simulink model "ev_battery_soc"  (R2026b)
settings: Solver=VariableStepAuto  StopTime=600
settings Model: Creator=Hassan  LastModifiedBy=Hassan

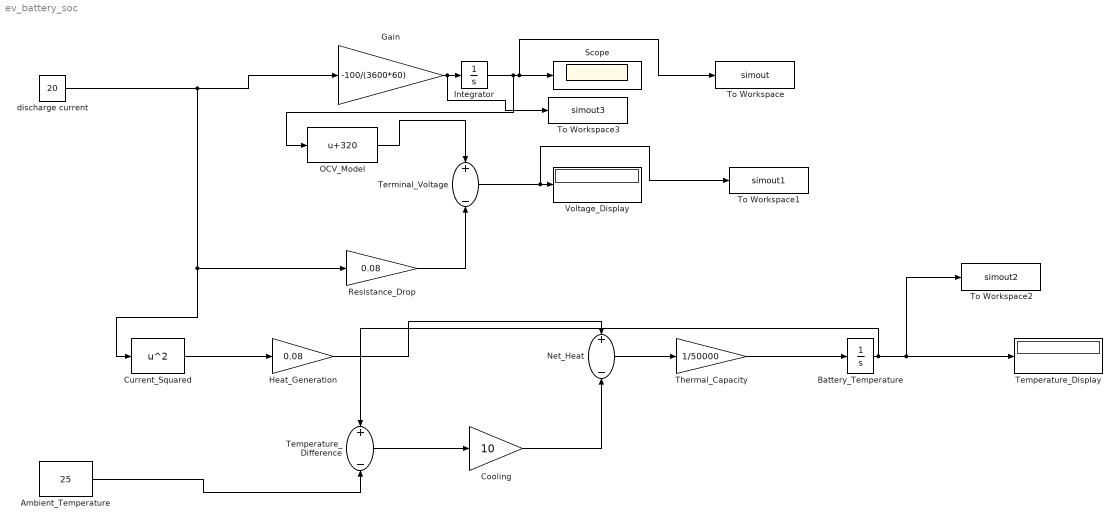
== system ev_battery_soc ==
  Ambient_Temperature : Constant  Value=25
  Battery_Temperature : Integrator  InitialCondition=25
  Cooling : Gain  Gain=10
  Current_Squared : Math  Operator=square
  Gain : Gain  Gain=-100/(3600*60)
  Heat_Generation : Gain  Gain=0.08
  Integrator : Integrator  InitialCondition=80
  Net_Heat : Sum  Inputs=+-
  OCV_Model : Bias  Bias=320  SaturateOnIntegerOverflow=off
  Resistance_Drop : Gain  Gain=0.08
  Scope : Scope
      settings: ActiveDisplayYMinimum=73.749999999999829  ActiveDisplayYMaximum=80.694444444444471
  Temperature_Difference : Sum  Inputs=+-
  Temperature_Display : Display
  Terminal_Voltage : Sum  Inputs=+-
  Thermal_Capacity : Gain  Gain=1/50000
  To Workspace : ToWorkspace  VariableName=simout  SaveFormat=Timeseries  SampleTime=-1
  To Workspace1 : ToWorkspace  VariableName=simout1  SaveFormat=Timeseries  SampleTime=-1
  To Workspace2 : ToWorkspace  VariableName=simout2  SaveFormat=Timeseries  SampleTime=-1
  To Workspace3 : ToWorkspace  VariableName=simout3  SaveFormat=Timeseries  SampleTime=-1
  Voltage_Display : Display
  discharge current : Constant  Value=20
  wires:
  Gain/1 -> To Workspace3/1, Integrator/1
  discharge current/1 -> Current_Squared/1, Resistance_Drop/1, Gain/1
  Integrator/1 -> OCV_Model/1, To Workspace/1, Scope/1
  OCV_Model/1 -> Terminal_Voltage/1
  Resistance_Drop/1 -> Terminal_Voltage/2
  Terminal_Voltage/1 -> To Workspace1/1, Voltage_Display/1
  Temperature_Difference/1 -> Cooling/1
  Current_Squared/1 -> Heat_Generation/1
  Heat_Generation/1 -> Net_Heat/1
  Cooling/1 -> Net_Heat/2
  Net_Heat/1 -> Thermal_Capacity/1
  Thermal_Capacity/1 -> Battery_Temperature/1
  Battery_Temperature/1 -> Temperature_Difference/1, To Workspace2/1, Temperature_Display/1
  Ambient_Temperature/1 -> Temperature_Difference/2
